simulink model "sm_car"  (R2025a)
settings: Solver=ode23t  StartTime=0.0  StopTime=400  MaxStep=0.4  RelTol=1e-3  AbsTol=1e-3  EnableMultiTasking=on
PreLoadFcn:
  | % Due to usability issue in Repeating Sequence block
  | warning('off','Simulink:Masking:Invalid');
  | 
  | % Eliminate unnecessary warnings in inactive variants
  | % Warnings generated only if you click through inactive variant
  | warning('off','MATLAB:nonExistentField');
  | warning('off','Simulink:Parameters:BlkParamUndefined');
PostLoadFcn:
  | set_param([bdroot '/Vehicle'],'popup_trailer','Off')
  | warning('off','sm:sli:setup:compile:LocalSolverNotSupported')
  | %sm_car_config_maneuver(bdroot,'WOT Braking');
  | sm_car_config_vehicle(bdroot,'false');
  | sm_car_config_logging(bdroot);
InitFcn:
  | sm_car_config_camera;
  | Vehicle = sm_car_vehcfg_checkConfig(Vehicle);
  | sm_car_check_tire_model(bdroot);
StartFcn:
  | tic;
StopFcn:
  | Elapsed_Sim_Time = toc;
  | % disp(['Elapsed Sim Time = ' num2str(Elapsed_Sim_Time)]);
undefined symbols (not defined in the file): Axle1D, AxleIn, Camera, Control, Driver, Free, Init, Maneuver, Pedal, RaceFix, RaceSpin, Scene, ShaftL1, ShaftL2, ShaftR1, ShaftR2, Soft, Stiff, Visual, X, xy_data_car_side, Y, Z
libraries: sm_lib x1546, nesl_utility x528, fl_lib x480, SimscapeFluids_lib x61, sdl_lib x49, simulink x29, ee_lib x7, simulink_extras x6, Linkage_Systems x4, Tire_1x2x x4, AntiRollBar_Systems x2, Linkage_Decoupled x2
(part 11 of 79)

== system sm_car/Vehicle/Vehicle/Chassis/SuspA1/Linkage Decoupled ==
  In Bus Element : Inport  PortName=CtrlBus  Element=Steer
  DrvBus : Inport  Port=2
  Linkage L : Linkage_Decoupled/Linkage  VariantControl=Variant1  LabelModeActiveChoice=DWDecoupled  popup_leftRight=Left  Linkage=Susp.Linkage  InitLinkage=Init  VariantLabel=Susp.Linkage.class.Value
      settings: AttributesFormatString=%<ActiveVariant>
  Linkage R : Linkage_Decoupled/Linkage  VariantControl=Variant1  LabelModeActiveChoice=DWDecoupled  popup_leftRight=Right  Linkage=Susp.Linkage  InitLinkage=Init  VariantLabel=Susp.Linkage.class.Value
      settings: AttributesFormatString=%<ActiveVariant>
  RollHeave Decouple : Subsystem  VariantControl=Variant1  mask(Roll and Heave Spring Dampers){hp_pushrod=Susp.Linkage.Pushrod.sBellcrank.Value, hp_bcr_pivot=Susp.Linkage.Bellcrank.sPivot.Value, hp_bcr_shock_heaveL=Susp.Linkage.Shock.Heave.sLeft.Value, hp_bcr_shock_heaveR=Susp.Linkage.Shock.Heave.sRight.Value, hp_bcr_shock_rollL=Susp.Linkage.Shock.Roll.sLeft.Value, hp_bcr_shock_rollR=Susp.Linkage.Shock.Roll.sRight.Value, shock_pist_mass_heave=Susp.Linkage.Shock.Heave.mPiston.Value, shock_pist_mass_roll=Susp.Linkage.Shock.Roll.mPiston.Value, shock_cyl_mass_heave=Susp.Linkage.Shock.Heave.mCylinder.Value, shock_cyl_mass_roll=Susp.Linkage.Shock.Roll.mCylinder.Value, up_lim_bumpstop_heave=Susp.Linkage.Endstop.Heave.xMax.Value, up_lim_bumpstop_roll=Susp.Linkage.Endstop.Roll.xMax.Value, low_lim_bumpstop_heave=Susp.Linkage.Endstop.Heave.xMin.Value, low_lim_bumpstop_roll=Susp.Linkage.Endstop.Roll.xMin.Value, clr_conn_shock=Visual.hp.clr, opc_conn_shock=Visual.hp.opc, size_conn_shock=Visual.hp.rad, clr_shock_cyl=Visual.Shock.cyl.clr, opc_shock_cyl=Visual.part.opc, radius_shock_cyl=Visual.Shock.cyl.rad, clr_shock_piston=Visual.Shock.piston.clr, opc_shock_piston=Visual.part.opc, clr_shock_bumpstop=Visual.Shock.bumpstop.clr, opc_shock_bumpstop=Visual.part.opc, deadvol_len_shock_cyl=Visual.Shock.dead_length, piston_len_shock=Visual.Shock.piston.len, cyl_cap_len_shock=Visual.Shock.cap.len, bumpstop_len_shock=Visual.Shock.bumpstop.len}
      mask prompts: hp_pushrod "HP Pushrod Inner  [xyz] (m)"; hp_bcr_pivot "HP Bellcrank Pivot [xyz] (m)"; deadvol_len_shock_cyl "Dead Volume Height (m)"; piston_len_shock "Piston Length (m)"; cyl_cap_len_shock "Cylinder Cap Length (m)"; bumpstop_len_shock "Bumpstop Length (m)"
      mask help: Models springs and dampers in a suspension design that decouples stiffness and damping for body roll and heave.
      mask init:
      | % Code to mirror hardpoint about vehicle xz plane
      | % and the plane defined by the bellcrank pivot axis
      | % and the y axis of the vehicle
      | % Code not used so that points can be specified independently
      | % Left here as a reference.
      | %{
      |  
      | a1 = atan2(hp_pushrod(1)-hp_bcr_pivot(1)   ,hp_pushrod(3)-hp_bcr_pivot(3));
      | a2 = atan2(hp_bcr_shock_roll(1)-hp_bcr_pivot(1),hp_bcr_shock_roll(3)-hp_bcr_pivot(3));
      | d_roll2piv = norm(hp_bcr_shock_roll([1 3])-hp_bcr_pivot([1 3]));
      | d_roll_mirror_axis = d_roll2piv*cos(a2-a1);
      | mirr_dx = d_roll_mirror_axis*sin(a1);
      | mirr_dz = d_roll_mirror_axis*cos(a1);
      | hp_bcr_shock_roll_r = ...
      |     [hp_bcr_shock_roll(1)-2*mirr_dx -hp_bcr_shock_roll(2) hp_bcr_shock_roll(3)-2*mirr_dz]
      | %}
      mask TypeOptions shock_pist_mass_heave: Shock Heave/shock_pist_mass
      mask TypeOptions shock_pist_mass_roll: Shock Roll/shock_pist_mass
      mask TypeOptions shock_cyl_mass_heave: Shock Heave/shock_cyl_mass
      mask TypeOptions shock_cyl_mass_roll: Shock Roll/shock_cyl_mass
      mask TypeOptions up_lim_bumpstop_heave: Shock Heave/up_lim_bumpstop
      mask TypeOptions up_lim_bumpstop_roll: Shock Roll/up_lim_bumpstop
      mask TypeOptions low_lim_bumpstop_heave: Shock Heave/low_lim_bumpstop
      mask TypeOptions low_lim_bumpstop_roll: Shock Roll/low_lim_bumpstop
      mask TypeOptions clr_conn_shock: Shock Heave/clr_conn_shock | Shock Roll/clr_conn_shock
      mask TypeOptions opc_conn_shock: Shock Heave/opc_conn_shock | Shock Roll/opc_conn_shock
      mask TypeOptions size_conn_shock: Shock Heave/size_conn_shock | Shock Roll/size_conn_shock
      mask TypeOptions clr_shock_cyl: Shock Heave/clr_shock_cyl | Shock Roll/clr_shock_cyl
      mask TypeOptions opc_shock_cyl: Shock Heave/opc_shock_cyl | Shock Roll/opc_shock_cyl
      mask TypeOptions radius_shock_cyl: Shock Heave/radius_shock_cyl | Shock Roll/radius_shock_cyl
      mask TypeOptions clr_shock_piston: Shock Heave/clr_shock_piston | Shock Roll/clr_shock_piston
      mask TypeOptions opc_shock_piston: Shock Heave/opc_shock_piston | Shock Roll/opc_shock_piston
      mask TypeOptions clr_shock_bumpstop: Shock Heave/clr_shock_bumpstop | Shock Roll/clr_shock_bumpstop
      mask TypeOptions opc_shock_bumpstop: Shock Heave/opc_shock_bumpstop | Shock Roll/opc_shock_bumpstop
      mask TypeOptions deadvol_len_shock_cyl: Shock Heave/deadvol_len_shock_cyl | Shock Roll/deadvol_len_shock_cyl
      mask TypeOptions piston_len_shock: Shock Heave/piston_len_shock | Shock Roll/piston_len_shock
      mask TypeOptions cyl_cap_len_shock: Shock Heave/cyl_cap_len_shock | Shock Roll/cyl_cap_len_shock
      mask TypeOptions bumpstop_len_shock: Shock Heave/bumpstop_len_shock | Shock Roll/bumpstop_len_shock
      mask DialogControl cont_hp Prompt: Hardpoints
      mask DialogControl text_hp_left Prompt: Left
      mask DialogControl text_hp_right Prompt: Right
      mask DialogControl text_hp_heave Prompt: Heave [xyz] (m)
      mask DialogControl text_hp_roll Prompt: Roll [xyz] (m)
      mask DialogControl cont_shock Prompt: Shock
      mask DialogControl text_shock_parts_blank Prompt: Parts
      mask DialogControl text_shock_heave Prompt: Heave
      mask DialogControl text_shock_roll Prompt: Roll
      mask DialogControl text_shock_pistm Prompt: Piston Mass (kg)
      mask DialogControl text_shock_cylm Prompt: Cylinder Mass (kg)
      mask DialogControl text_shock_bumpstop_par Prompt: Bumpstop
      mask DialogControl text_bump_ul Prompt: Upper Limit (m)
      mask DialogControl text_bump_low Prompt: Lower Limit (m)
      mask DialogControl cont_vis_shock Prompt: Visualization
      mask DialogControl text_clr_shock Prompt: Color  [RGB]
      mask DialogControl text_opc_shock Prompt: Opac. (0-1)
      mask DialogControl text_size_shock Prompt: Size (m)
      mask DialogControl text_conn_shock Prompt: Connections
      mask DialogControl text_shock_shock Prompt: Cylinder
      mask DialogControl text_shock_piston Prompt: Piston
      mask DialogControl text_piston_radius Prompt: <cylinder radius>
      mask DialogControl text_shock_bumpstop Prompt: Bumpstop
      mask DialogControl text_bumpstop_radius Prompt: <cylinder radius>
      mask Display: image('sm_car_vehicle_linkage_rollHeaveDecouple_IMAGE.png');
  Simscape Bus L : SimscapeBus  HierarchyStrings=RaceSpin;RaceFix;Axle1D;AxleIn
  Simscape Bus L1 : SimscapeBus  HierarchyStrings=RaceSpin;RaceFix;Axle1D;AxleIn
  Steer : Subsystem  Variant=on  VariantControlMode=label  VariantControl=Steer  LabelModeActiveChoice=WheelDrivenRack1UJoint  mask(Steering System with Rack){Steer=Susp.Steer, VariantLabel=Susp.Steer.class.Value}
      mask prompts: Steer "Steer Parameters"; VariantLabel "Variant Label"
      mask help: Models steering system that involves a rack. Optionally include steering wheel. Connection between steering wheel and rack can be mechanical, specified by a lookup table, or a control system as in steer-by-wire. Option is chosen by string provided in Variant Label. The parameters for the selected option are contained in Steer data structure.
      mask init:
      | curblk = gcb;
      | 
      | % Set variant for this block 
      | set_param(curblk,'LabelModeActiveChoice',VariantLabel);
      settings: AttributesFormatString=%<ActiveVariant>
      mask Display: disp(' ');
  Wheel Meas Left : Subsystem  mask(Wheel Measurements){popup_leftRight=Left}
      mask prompts: popup_leftRight "Left/Right"
      mask help: Calculates toe and camber angles based on orientation of wheel spin axis. To estimate steering axis inclination, the same measurements are done along the longitudinal axis (X) of the tire. Set Left/Right so that the sign of the logged toe and camber angles is associated with towards/away from vehicle center.
      mask init:
      | if(popup_leftRight == 1)
      |     rhs_tc = 1;
      | elseif(popup_leftRight == 2)
      |     rhs_tc = -1;
      | end
      mask TypeOptions popup_leftRight: Left | Right
  Wheel Meas Right : Subsystem  mask(Wheel Measurements){popup_leftRight=Right}
      mask prompts: popup_leftRight "Left/Right"
      mask help: Calculates toe and camber angles based on orientation of wheel spin axis. To estimate steering axis inclination, the same measurements are done along the longitudinal axis (X) of the tire. Set Left/Right so that the sign of the logged toe and camber angles is associated with towards/away from vehicle center.
      mask init:
      | if(popup_leftRight == 1)
      |     rhs_tc = 1;
      | elseif(popup_leftRight == 2)
      |     rhs_tc = -1;
      | end
      mask TypeOptions popup_leftRight: Left | Right
  WCL : PMIOPort  Side=Left
  Ref : PMIOPort  Port=2  Side=Right
  WCR : PMIOPort  Port=3  Side=Right
  AxleL : PMIOPort  Port=4  Side=Left
  AxleR : PMIOPort  Port=5  Side=Right
  SprL : PMIOPort  Port=6  Side=Left
  SprR : PMIOPort  Port=7  Side=Right
  DmpL : PMIOPort  Port=8  Side=Left
  DmpR : PMIOPort  Port=9  Side=Right
  Out Bus Element : Outport  VectorParamsAs1DForOutWhenUnconnected=off  PortName=OutBus  Element=Steer
  Out Bus Element1 : Outport  VectorParamsAs1DForOutWhenUnconnected=off  PortName=OutBus  Element=RollHeave
  Out Bus Element2 : Outport  VectorParamsAs1DForOutWhenUnconnected=off  PortName=OutBus  Element=WhlL
  Out Bus Element3 : Outport  VectorParamsAs1DForOutWhenUnconnected=off  PortName=OutBus  Element=WhlR
  Out Bus Element4 : Outport  VectorParamsAs1DForOutWhenUnconnected=off  PortName=OutBus  Element=LinkageR
  Out Bus Element5 : Outport  VectorParamsAs1DForOutWhenUnconnected=off  PortName=OutBus  Element=LinkageL
  wires:
  Linkage L/1 -> Out Bus Element5/1
  Linkage R/1 -> Out Bus Element4/1
  RollHeave Decouple/1(meas) -> Out Bus Element1/1
  DrvBus/1 -> Steer/1(DrvBus)
  Steer/1(" meas") -> Out Bus Element/1
  In Bus Element/1 -> Steer/2(CtrlBus)
  Wheel Meas Left/1(meas) -> Out Bus Element2/1
  Wheel Meas Right/1(meas) -> Out Bus Element3/1
  connections:
  SprR/RConn1 -- RollHeave Decouple/LConn5
  DmpR/RConn1 -- RollHeave Decouple/LConn6
  SprL/RConn1 -- RollHeave Decouple/LConn3
  DmpL/RConn1 -- RollHeave Decouple/LConn4
  RollHeave Decouple/LConn8 -- Linkage R/LConn6
  RollHeave Decouple/LConn7 -- Linkage R/LConn7
  RollHeave Decouple/LConn2 -- Linkage L/LConn7
  Steer/RConn3 -- Linkage R/RConn1
  Linkage L/RConn2 -- Ref/RConn1 -- Linkage R/RConn2 -- Wheel Meas Left/LConn1 -- Wheel Meas Right/LConn1 -- Steer/RConn2
  WCL/RConn1 -- Linkage L/LConn1 -- Wheel Meas Left/LConn2
  WCR/RConn1 -- Linkage R/LConn1 -- Wheel Meas Right/LConn2
  Steer/RConn1 -- Linkage L/RConn1
  Linkage L/LConn5 -- Simscape Bus L/LConn4
  Linkage L/LConn2 -- Simscape Bus L/LConn1
  Linkage L/LConn3 -- Simscape Bus L/LConn2
  Linkage L/LConn4 -- Simscape Bus L/LConn3
  AxleL/RConn1 -- Simscape Bus L/RConn1
  Linkage R/LConn2 -- Simscape Bus L1/LConn1
  Linkage R/LConn3 -- Simscape Bus L1/LConn2
  Linkage R/LConn4 -- Simscape Bus L1/LConn3
  Simscape Bus L1/RConn1 -- AxleR/RConn1
  Linkage R/LConn5 -- Simscape Bus L1/LConn4
  RollHeave Decouple/LConn1 -- Linkage L/LConn6

== system sm_car/Vehicle/Vehicle/Chassis/SuspA2/Linkage ==
  In Bus Element : Inport  PortName=CtrlBus  Element=Steer
  DrvBus : Inport  Port=2
  Anti Roll Bar : AntiRollBar_Systems/Anti Roll Bar  LabelModeActiveChoice=DroplinkRod  AntiRollBar=Susp.AntiRollBar  VariantLabel=Susp.AntiRollBar.class.Value
      settings: AttributesFormatString=%<LabelModeActiveChoice>
  Linkage L : Linkage_Systems/Linkage  VariantControl=Variant1  LabelModeActiveChoice=DoubleWishboneA  popup_leftRight=Left  Linkage=Susp.Linkage  InitLinkage=Init  VariantLabel=Susp.Linkage.class.Value
      settings: AttributesFormatString=%<ActiveVariant>
  Linkage R : Linkage_Systems/Linkage  Tag=PublishSubsystem  VariantControl=Variant1  LabelModeActiveChoice=DoubleWishboneA  popup_leftRight=Right  Linkage=Susp.Linkage  InitLinkage=Init  VariantLabel=Susp.Linkage.class.Value
      settings: AttributesFormatString=%<ActiveVariant>
  Simscape Bus L : SimscapeBus  HierarchyStrings=RaceSpin;RaceFix;Axle1D;AxleIn
  Simscape Bus L1 : SimscapeBus  HierarchyStrings=RaceSpin;RaceFix;Axle1D;AxleIn
  Steer : Subsystem  Variant=on  VariantControlMode=label  VariantControl=Steer  LabelModeActiveChoice=None  mask(Steering System with Rack){Steer=Susp.Steer, VariantLabel=Susp.Steer.class.Value}
      mask prompts: Steer "Steer Parameters"; VariantLabel "Variant Label"
      mask help: Models steering system that involves a rack. Optionally include steering wheel. Connection between steering wheel and rack can be mechanical, specified by a lookup table, or a control system as in steer-by-wire. Option is chosen by string provided in Variant Label. The parameters for the selected option are contained in Steer data structure.
      mask init:
      | curblk = gcb;
      | 
      | % Set variant for this block 
      | set_param(curblk,'LabelModeActiveChoice',VariantLabel);
      settings: AttributesFormatString=%<ActiveVariant>
      mask Display: disp(' ');
  Wheel Meas Left : Subsystem  mask(Wheel Measurements){popup_leftRight=Left}
      mask prompts: popup_leftRight "Left/Right"
      mask help: Calculates toe and camber angles based on orientation of wheel spin axis. To estimate steering axis inclination, the same measurements are done along the longitudinal axis (X) of the tire. Set Left/Right so that the sign of the logged toe and camber angles is associated with towards/away from vehicle center.
      mask init:
      | if(popup_leftRight == 1)
      |     rhs_tc = 1;
      | elseif(popup_leftRight == 2)
      |     rhs_tc = -1;
      | end
      mask TypeOptions popup_leftRight: Left | Right
  Wheel Meas Right : Subsystem  mask(Wheel Measurements){popup_leftRight=Right}
      mask prompts: popup_leftRight "Left/Right"
      mask help: Calculates toe and camber angles based on orientation of wheel spin axis. To estimate steering axis inclination, the same measurements are done along the longitudinal axis (X) of the tire. Set Left/Right so that the sign of the logged toe and camber angles is associated with towards/away from vehicle center.
      mask init:
      | if(popup_leftRight == 1)
      |     rhs_tc = 1;
      | elseif(popup_leftRight == 2)
      |     rhs_tc = -1;
      | end
      mask TypeOptions popup_leftRight: Left | Right
  WCL : PMIOPort  Side=Left
  Ref : PMIOPort  Port=2  Side=Right
  WCR : PMIOPort  Port=3  Side=Right
  AxleL : PMIOPort  Port=4  Side=Left
  AxleR : PMIOPort  Port=5  Side=Right
  SprL : PMIOPort  Port=6  Side=Left
  SprR : PMIOPort  Port=7  Side=Right
  DmpL : PMIOPort  Port=8  Side=Left
  DmpR : PMIOPort  Port=9  Side=Right
  Out Bus Element : Outport  VectorParamsAs1DForOutWhenUnconnected=off  PortName=OutBus  Element=Steer
  Out Bus Element1 : Outport  VectorParamsAs1DForOutWhenUnconnected=off  PortName=OutBus  Element=AntiRollBar
  Out Bus Element2 : Outport  VectorParamsAs1DForOutWhenUnconnected=off  PortName=OutBus  Element=WhlL
  Out Bus Element3 : Outport  VectorParamsAs1DForOutWhenUnconnected=off  PortName=OutBus  Element=WhlR
  Out Bus Element4 : Outport  VectorParamsAs1DForOutWhenUnconnected=off  PortName=OutBus  Element=LinkageR
  Out Bus Element5 : Outport  VectorParamsAs1DForOutWhenUnconnected=off  PortName=OutBus  Element=LinkageL
  wires:
  Linkage L/1 -> Out Bus Element5/1
  Linkage R/1 -> Out Bus Element4/1
  DrvBus/1 -> Steer/1(DrvBus)
  Steer/1(" meas") -> Out Bus Element/1
  In Bus Element/1 -> Steer/2(CtrlBus)
  Anti Roll Bar/1 -> Out Bus Element1/1
  Wheel Meas Left/1(meas) -> Out Bus Element2/1
  Wheel Meas Right/1(meas) -> Out Bus Element3/1
  connections:
  Steer/RConn3 -- Linkage R/RConn1
  Ref/RConn1 -- Anti Roll Bar/LConn2 -- Linkage R/RConn2 -- Wheel Meas Right/LConn1 -- Wheel Meas Left/LConn1 -- Steer/RConn2 -- Linkage L/RConn2
  Linkage L/LConn1 -- WCL/RConn1 -- Wheel Meas Left/LConn2
  Linkage R/LConn1 -- WCR/RConn1 -- Wheel Meas Right/LConn2
  Steer/RConn1 -- Linkage L/RConn1
  DmpL/RConn1 -- Linkage L/LConn7
  Simscape Bus L/LConn4 -- Linkage L/LConn5
  Simscape Bus L/LConn1 -- Linkage L/LConn2
  Linkage L/LConn3 -- Simscape Bus L/LConn2
  Linkage L/LConn4 -- Simscape Bus L/LConn3
  AxleL/RConn1 -- Simscape Bus L/RConn1
  DmpR/RConn1 -- Linkage R/LConn7
  SprR/RConn1 -- Linkage R/LConn6
  Simscape Bus L1/LConn1 -- Linkage R/LConn2
  Simscape Bus L1/LConn2 -- Linkage R/LConn3
  Simscape Bus L1/LConn3 -- Linkage R/LConn4
  Simscape Bus L1/RConn1 -- AxleR/RConn1
  SprL/RConn1 -- Linkage L/LConn6
  Simscape Bus L1/LConn4 -- Linkage R/LConn5
  Anti Roll Bar/LConn3 -- Linkage R/LConn8
  Anti Roll Bar/LConn1 -- Linkage L/LConn8

== system sm_car/Vehicle/Vehicle/Powertrain/Driveline/L1 R1 L2 R2 ==
  note: Port
      | placement
  In Bus Element1 : Inport  PortName=CtrlBus
  Gearbox L1 : sdl_lib/Gears/Simple Gear  ratio=Driveline.GearboxL1.ratio.Value  rotation_direction=3-2*(1)  friction_model=1  T_noload=0.1 N*m  T_nom=5 N*m  efficiency_nom=0.8  efficiency=0.8  temperature_TLU=[280, 300, 320] K  load_TLU=[1, 5, 10] N*m  efficiency_TLU=[.95, .9, .85]  efficiency_TLU2=[.85, .8, .75; .95, .9, .85; .85, .8, .7]  w_thr=0.01 rad/s  pwr_thr=0.001 W  enable_backlash=false  hardstop_model=simscape.enum.hardstop.smooth  backlash_distance=1e-3 mm  r_base=0.1 m  transition=1e-4 mm  backlash_stiffness=1e7 N/m  backlash_damping=1e6 N*s/m  coeff_rest=0  v_tol=0.001 m/s  f_tol=0 N  mu_visc=[0, 0] N*m/(rad/s)  thermal_mass=50 J/K  temperature_specify=off  temperature_priority=High  temperature=300 K  temperature_nominal_specify=off  temperature_nominal_value=1  temperature_nominal_unit=K  x_backlash_specify=off  x_backlash_priority=None  x_backlash=0 mm  x_backlash_nominal_specify=off  x_backlash_nominal_value=1  x_backlash_nominal_unit=mm  f_hardstop_specify=off  f_hardstop_priority=None  f_hardstop=0 N  f_hardstop_nominal_specify=off  f_hardstop_nominal_value=1  f_hardstop_nominal_unit=N  v_backlash_specify=off  v_backlash_priority=None  v_backlash=0 m/s  v_backlash_nominal_specify=off  v_backlash_nominal_value=1  v_backlash_nominal_unit=m/s
  Gearbox L2 : sdl_lib/Gears/Simple Gear  ratio=Driveline.GearboxL2.ratio.Value  rotation_direction=3-2*(1)  friction_model=1  T_noload=0.1 N*m  T_nom=5 N*m  efficiency_nom=0.8  efficiency=0.8  temperature_TLU=[280, 300, 320] K  load_TLU=[1, 5, 10] N*m  efficiency_TLU=[.95, .9, .85]  efficiency_TLU2=[.85, .8, .75; .95, .9, .85; .85, .8, .7]  w_thr=0.01 rad/s  pwr_thr=0.001 W  enable_backlash=false  hardstop_model=simscape.enum.hardstop.smooth  backlash_distance=1e-3 mm  r_base=0.1 m  transition=1e-4 mm  backlash_stiffness=1e7 N/m  backlash_damping=1e6 N*s/m  coeff_rest=0  v_tol=0.001 m/s  f_tol=0 N  mu_visc=[0, 0] N*m/(rad/s)  thermal_mass=50 J/K  temperature_specify=off  temperature_priority=High  temperature=300 K  temperature_nominal_specify=off  temperature_nominal_value=1  temperature_nominal_unit=K  x_backlash_specify=off  x_backlash_priority=None  x_backlash=0 mm  x_backlash_nominal_specify=off  x_backlash_nominal_value=1  x_backlash_nominal_unit=mm  f_hardstop_specify=off  f_hardstop_priority=None  f_hardstop=0 N  f_hardstop_nominal_specify=off  f_hardstop_nominal_value=1  f_hardstop_nominal_unit=N  v_backlash_specify=off  v_backlash_priority=None  v_backlash=0 m/s  v_backlash_nominal_specify=off  v_backlash_nominal_value=1  v_backlash_nominal_unit=m/s
  Gearbox R1 : sdl_lib/Gears/Simple Gear  ratio=Driveline.GearboxL1.ratio.Value  rotation_direction=3-2*(1)  friction_model=1  T_noload=0.1 N*m  T_nom=5 N*m  efficiency_nom=0.8  efficiency=0.8  temperature_TLU=[280, 300, 320] K  load_TLU=[1, 5, 10] N*m  efficiency_TLU=[.95, .9, .85]  efficiency_TLU2=[.85, .8, .75; .95, .9, .85; .85, .8, .7]  w_thr=0.01 rad/s  pwr_thr=0.001 W  enable_backlash=false  hardstop_model=simscape.enum.hardstop.smooth  backlash_distance=1e-3 mm  r_base=0.1 m  transition=1e-4 mm  backlash_stiffness=1e7 N/m  backlash_damping=1e6 N*s/m  coeff_rest=0  v_tol=0.001 m/s  f_tol=0 N  mu_visc=[0, 0] N*m/(rad/s)  thermal_mass=50 J/K  temperature_specify=off  temperature_priority=High  temperature=300 K  temperature_nominal_specify=off  temperature_nominal_value=1  temperature_nominal_unit=K  x_backlash_specify=off  x_backlash_priority=None  x_backlash=0 mm  x_backlash_nominal_specify=off  x_backlash_nominal_value=1  x_backlash_nominal_unit=mm  f_hardstop_specify=off  f_hardstop_priority=None  f_hardstop=0 N  f_hardstop_nominal_specify=off  f_hardstop_nominal_value=1  f_hardstop_nominal_unit=N  v_backlash_specify=off  v_backlash_priority=None  v_backlash=0 m/s  v_backlash_nominal_specify=off  v_backlash_nominal_value=1  v_backlash_nominal_unit=m/s
  Gearbox R2 : sdl_lib/Gears/Simple Gear  ratio=Driveline.GearboxR2.ratio.Value  rotation_direction=3-2*(1)  friction_model=1  T_noload=0.1 N*m  T_nom=5 N*m  efficiency_nom=0.8  efficiency=0.8  temperature_TLU=[280, 300, 320] K  load_TLU=[1, 5, 10] N*m  efficiency_TLU=[.95, .9, .85]  efficiency_TLU2=[.85, .8, .75; .95, .9, .85; .85, .8, .7]  w_thr=0.01 rad/s  pwr_thr=0.001 W  enable_backlash=false  hardstop_model=simscape.enum.hardstop.smooth  backlash_distance=1e-3 mm  r_base=0.1 m  transition=1e-4 mm  backlash_stiffness=1e7 N/m  backlash_damping=1e6 N*s/m  coeff_rest=0  v_tol=0.001 m/s  f_tol=0 N  mu_visc=[0, 0] N*m/(rad/s)  thermal_mass=50 J/K  temperature_specify=off  temperature_priority=High  temperature=300 K  temperature_nominal_specify=off  temperature_nominal_value=1  temperature_nominal_unit=K  x_backlash_specify=off  x_backlash_priority=None  x_backlash=0 mm  x_backlash_nominal_specify=off  x_backlash_nominal_value=1  x_backlash_nominal_unit=mm  f_hardstop_specify=off  f_hardstop_priority=None  f_hardstop=0 N  f_hardstop_nominal_specify=off  f_hardstop_nominal_value=1  f_hardstop_nominal_unit=N  v_backlash_specify=off  v_backlash_priority=None  v_backlash=0 m/s  v_backlash_nominal_specify=off  v_backlash_nominal_value=1  v_backlash_nominal_unit=m/s
  Reference Frame : sm_lib/Frames and Transforms/Reference Frame
  Reference Frame1 : sm_lib/Frames and Transforms/Reference Frame
  Sensing Torque L1 : Subsystem
  Sensing Torque L2 : Subsystem
  Sensing Torque R1 : Subsystem
  Sensing Torque R2 : Subsystem
  ShaftL1 : Subsystem  VariantControl=Shaft1D  mask(Driveshaft Assembly (1D)){}
      mask help: Models a shaft as a 1D mechanical connection.
  ShaftL2 : Subsystem  VariantControl=Shaft1D  mask(Driveshaft Assembly (1D)){}
      mask help: Models a shaft as a 1D mechanical connection.
  ShaftR1 : Subsystem  VariantControl=Shaft1D  mask(Driveshaft Assembly (1D)){}
      mask help: Models a shaft as a 1D mechanical connection.
  ShaftR2 : Subsystem  VariantControl=Shaft1D  mask(Driveshaft Assembly (1D)){}
      mask help: Models a shaft as a 1D mechanical connection.
  Simscape Bus : SimscapeBus  HierarchyStrings=ShaftL1;ShaftR1;ShaftR2;ShaftL2
  Simscape L1 : SimscapeBus  HierarchyStrings=Shaft1D
  Simscape L2 : SimscapeBus  HierarchyStrings=Shaft1D
  Simscape R1 : SimscapeBus  HierarchyStrings=Shaft1D
  Simscape R2 : SimscapeBus  HierarchyStrings=Shaft1D
  Terminator : Terminator
  A1 : PMIOPort  Side=Left
  A2 : PMIOPort  Port=2  Side=Right
  L1 : PMIOPort  Port=3  Side=Left
  R1 : PMIOPort  Port=4  Side=Right
  L2 : PMIOPort  Port=5  Side=Left
  R2 : PMIOPort  Port=6  Side=Right
  Shafts : PMIOPort  Port=7  Side=Left
  o : PMIOPort  Port=8  Side=Right
  Out Bus Element6 : Outport  VectorParamsAs1DForOutWhenUnconnected=off  PortName=OutD  Element=MDriveshaftL2
  Out Bus Element7 : Outport  VectorParamsAs1DForOutWhenUnconnected=off  PortName=OutD  Element=MDriveshaftR2
  Out Bus Element4 : Outport  VectorParamsAs1DForOutWhenUnconnected=off  PortName=OutD  Element=MDriveshaftR1
  Out Bus Element5 : Outport  VectorParamsAs1DForOutWhenUnconnected=off  PortName=OutD  Element=MDriveshaftL1
  Out Bus Element : Outport  VectorParamsAs1DForOutWhenUnconnected=off  PortName=OutD  Element=anDriveshaftL1
  Out Bus Element1 : Outport  VectorParamsAs1DForOutWhenUnconnected=off  PortName=OutD  Element=anDriveshaftR1
  Out Bus Element2 : Outport  VectorParamsAs1DForOutWhenUnconnected=off  PortName=OutD  Element=anDriveshaftL2
  Out Bus Element3 : Outport  VectorParamsAs1DForOutWhenUnconnected=off  PortName=OutD  Element=anDriveshaftR2
  wires:
  ShaftR1/1(meas) -> Out Bus Element1/1
  ShaftL1/1(meas) -> Out Bus Element/1
  ShaftL2/1(meas) -> Out Bus Element2/1
  ShaftR2/1(meas) -> Out Bus Element3/1
  Sensing Torque R2/1(M) -> Out Bus Element7/1
  Sensing Torque L2/1(M) -> Out Bus Element6/1
  Sensing Torque R1/1(M) -> Out Bus Element4/1
  Sensing Torque L1/1(M) -> Out Bus Element5/1
  In Bus Element1/1 -> Terminator/1
  connections:
  Gearbox L2/RConn1 -- Sensing Torque L2/LConn1
  Sensing Torque R2/LConn1 -- Gearbox R2/RConn1
  Simscape L1/LConn1 -- Sensing Torque L1/RConn1
  Sensing Torque R1/RConn1 -- Simscape R1/LConn1
  Sensing Torque R1/LConn1 -- Gearbox R1/RConn1
  Gearbox R1/LConn1 -- Simscape Bus/LConn2 -- o/RConn1
  A1/RConn1 -- Reference Frame1/RConn1
  ShaftL1/RConn1 -- Simscape L1/RConn1
  Gearbox L1/RConn1 -- Sensing Torque L1/LConn1
  Simscape Bus/LConn3 -- Gearbox R2/LConn1
  Gearbox L2/LConn1 -- Simscape Bus/LConn4
  Simscape L2/LConn1 -- Sensing Torque L2/RConn1
  Simscape L2/RConn1 -- ShaftL2/RConn1
  Gearbox L1/LConn1 -- Simscape Bus/LConn1
  ShaftR1/RConn1 -- Simscape R1/RConn1
  ShaftR1/LConn1 -- R1/RConn1
  ShaftL1/LConn1 -- L1/RConn1
  Reference Frame/RConn1 -- A2/RConn1
  ShaftR2/LConn1 -- R2/RConn1
  ShaftL2/LConn1 -- L2/RConn1
  Simscape R2/RConn1 -- ShaftR2/RConn1
  Sensing Torque R2/RConn1 -- Simscape R2/LConn1
  Simscape Bus/RConn1 -- Shafts/RConn1

== system sm_car/Vehicle/Vehicle/Powertrain/Power/Electric L1 R1 L2 R2 ==
  note: Future:
      | react torque
      | from drive
      | on chassis
  In Bus Element1 : Inport  PortName=CtrlBus  Element=MMotorL1Demand
  In Bus Element2 : Inport  PortName=CtrlBus  Element=MMotorL2Demand
  In Bus Element3 : Inport  PortName=CtrlBus  Element=MMotorR2Demand
  In Bus Element4 : Inport  PortName=CtrlBus  Element=MMotorR1Demand
  VehBus : Inport  Port=2
  Ambient Temperature : fl_lib/Thermal/Thermal Sources/Temperature Source  temperature=Power.TAmbient.Value K
  Battery : Subsystem
      mask Display: image('sm_car_vehicle_power_battery_system_IMAGE.png');
  ERef DC Bus : fl_lib/Electrical/Electrical Elements/Electrical Reference
  Motor L1 : Subsystem  mask(Motor and Drive){Motor=Power.MotorL1}
      mask prompts: Motor "Motor (Structure)"
      mask help: Models generic motor and drive with closed-loop torque control. Specify torque-speed curve and other parameters in the Motor data structure.
      mask Display: image('sm_car_vehicle_power_emotor_simplified_IMAGE.png');
  Motor L2 : Subsystem  mask(Motor and Drive){Motor=Power.MotorL2}
      mask prompts: Motor "Motor (Structure)"
      mask help: Models generic motor and drive with closed-loop torque control. Specify torque-speed curve and other parameters in the Motor data structure.
      mask Display: image('sm_car_vehicle_power_emotor_simplified_IMAGE.png');
  Motor R1 : Subsystem  mask(Motor and Drive){Motor=Power.MotorL1}
      mask prompts: Motor "Motor (Structure)"
      mask help: Models generic motor and drive with closed-loop torque control. Specify torque-speed curve and other parameters in the Motor data structure.
      mask Display: image('sm_car_vehicle_power_emotor_simplified_IMAGE.png');
  Motor R2 : Subsystem  mask(Motor and Drive){Motor=Power.MotorL2}
      mask prompts: Motor "Motor (Structure)"
      mask help: Models generic motor and drive with closed-loop torque control. Specify torque-speed curve and other parameters in the Motor data structure.
      mask Display: image('sm_car_vehicle_power_emotor_simplified_IMAGE.png');
  Reference Frame : sm_lib/Frames and Transforms/Reference Frame
  Simscape Bus : SimscapeBus  HierarchyStrings=ShaftL1;ShaftR1;ShaftL2;ShaftR2
  Terminator : Terminator
  Thermal : Subsystem  Variant=on  VariantControlMode=label  VariantControl=Variant1  LabelModeActiveChoice=Liquid_Loop1  mask(Variants for Cooling System){VariantLabel=Power.Cooling.class.Value}
      mask prompts: VariantLabel "Variant Label"
      mask help: Select option and provide parameters for cooling system. Option is chosen by string provided in Variant Label.
      mask init:
      | curblk = gcb;
      | 
      | % Set variant for this block 
      | set_param(curblk,'LabelModeActiveChoice',VariantLabel);
      settings: AttributesFormatString=%<ActiveVariant>
  Shafts : PMIOPort  Side=Left
  Ref : PMIOPort  Port=2  Side=Right
  Out Bus Element : Outport  VectorParamsAs1DForOutWhenUnconnected=off  PortName=OutP  Element=MotorL2
  Out Bus Element1 : Outport  VectorParamsAs1DForOutWhenUnconnected=off  PortName=OutP  Element=MotorR2
  Out Bus Element2 : Outport  VectorParamsAs1DForOutWhenUnconnected=off  PortName=OutP  Element=MotorL1
  Out Bus Element3 : Outport  VectorParamsAs1DForOutWhenUnconnected=off  PortName=OutP  Element=Thermal
  Out Bus Element4 : Outport  VectorParamsAs1DForOutWhenUnconnected=off  PortName=OutP  Element=Battery
  Out Bus Element5 : Outport  VectorParamsAs1DForOutWhenUnconnected=off  PortName=OutP  Element=MotorR1
  wires:
  In Bus Element4/1 -> Motor R1/1(Tr)
  Motor R1/1(m) -> Out Bus Element5/1
  Battery/1(m) -> Out Bus Element4/1
  VehBus/1 -> Terminator/1
  Thermal/1(" m") -> Out Bus Element3/1
  In Bus Element3/1 -> Motor R2/1(Tr)
  Motor L1/1(m) -> Out Bus Element2/1
  Motor R2/1(m) -> Out Bus Element1/1
  Motor L2/1(m) -> Out Bus Element/1
  In Bus Element1/1 -> Motor L1/1(Tr)
  In Bus Element2/1 -> Motor L2/1(Tr)
  connections:
  Motor R1/LConn3 -- Thermal/LConn3
  Motor R1/RConn1 -- Simscape Bus/LConn2
  Thermal/RConn1 -- Battery/LConn1
  Battery/RConn3 -- Thermal/LConn1
  Thermal/RConn2 -- Ambient Temperature/LConn1
  Motor R2/LConn3 -- Thermal/LConn5
  Motor L2/LConn3 -- Thermal/LConn4
  Motor L1/LConn3 -- Thermal/LConn2
  Ref/RConn1 -- Reference Frame/RConn1
  Simscape Bus/RConn1 -- Shafts/RConn1
  Motor L2/RConn1 -- Simscape Bus/LConn3
  Motor L1/RConn1 -- Simscape Bus/LConn1
  Motor R2/LConn1 -- Motor L1/LConn1 -- Battery/RConn1 -- Motor R1/LConn1 -- Motor L2/LConn1
  Motor L1/LConn2 -- Battery/RConn2 -- Motor R1/LConn2 -- ERef DC Bus/LConn1 -- Motor R2/LConn2 -- Motor L2/LConn2
  Motor R2/RConn1 -- Simscape Bus/LConn4

== system sm_car/World/Scene/CRG Hockenheim/Finish Line/L1 ==
  Square LL : sm_lib/Body Elements/Brick Solid  BrickDimensions=square_lwh  BrickDimensionsUnits=m  ExportEntireGeometry=off  InertiaType=CalculateFromGeometry  BasedOnType=Density  Density=1000  DensityUnits=kg/m^3  Mass=1  MassUnits=kg  CenterOfMass=[0 0 0]  CenterOfMassUnits=m  MomentsOfInertia=[1 1 1]  MomentsOfInertiaUnits=kg*m^2  ProductsOfInertia=[0 0 0]  ProductsOfInertiaUnits=kg*m^2  GraphicType=FromGeometry  MarkerShape=Sphere  MarkerSize=10  GraphicVisPropType=SimpleVisualProperties  GraphicDiffuseColor=[0.0 0.0 0.0]  GraphicOpacity=1.0  GraphicSpecularColor=[0.5 0.5 0.5 1.0]  GraphicAmbientColor=[0.15 0.15 0.15 1.0]  GraphicEmissiveColor=[0.0 0.0 0.0 1.0]  GraphicShininess=75  DoExposeReferenceFrame=off  SerializedFrames=<Frames><Frame><Id>Frame1</Id><Value><Name>BL</Name><Origin><Source>GeometricFeature</Source><FeatureName>+y -z curve</FeatureName></Origin><PrimaryAxis><DefinedDirection>+Z</DefinedDirection><Source>ReferenceFrame</Source><SourceDirection>+Z</SourceDirection><FeatureName></FeatureName></PrimaryAxis><SecondaryAxis><DefinedDirection>+X</DefinedDirection><Source>ReferenceFrame</Source><SourceDirection>+X</SourceDirection><FeatureName></FeatureName></SecondaryAxis></Value></Frame><Frame><Id>Frame2</Id><Value><Name>TL</Name><Origin><Source>GeometricFeature</Source><FeatureName>+x +y +z point</FeatureName></Origin><PrimaryAxis><DefinedDirection>+Z</DefinedDirection><Source>ReferenceFrame</Source><SourceDirection>+Z</SourceDirection><FeatureName></FeatureName></PrimaryAxis><SecondaryAxis><DefinedDirection>+X</DefinedDirection><Source>ReferenceFrame</Source><SourceDirection>+X</SourceDirection><FeatureName></FeatureName></SecondaryAxis></Value></Frame><Frame><Id>Frame3</Id><Value><Name>BR</Name><Origin><Source>GeometricFeature</Source><FeatureName>-y -z curve</FeatureName></Origin><PrimaryAxis><DefinedDirection>+Z</DefinedDirection><Source>ReferenceFrame</Source><SourceDirection>+Z</SourceDirection><FeatureName></FeatureName></PrimaryAxis><SecondaryAxis><DefinedDirection>+X</DefinedDirection><Source>ReferenceFrame</Source><SourceDirection>+X</SourceDirection><FeatureName></FeatureName></SecondaryAxis></Value></Frame></Frames>
  Square LR : sm_lib/Body Elements/Brick Solid  BrickDimensions=square_lwh  BrickDimensionsUnits=m  ExportEntireGeometry=off  InertiaType=CalculateFromGeometry  BasedOnType=Density  Density=1000  DensityUnits=kg/m^3  Mass=1  MassUnits=kg  CenterOfMass=[0 0 0]  CenterOfMassUnits=m  MomentsOfInertia=[1 1 1]  MomentsOfInertiaUnits=kg*m^2  ProductsOfInertia=[0 0 0]  ProductsOfInertiaUnits=kg*m^2  GraphicType=FromGeometry  MarkerShape=Sphere  MarkerSize=10  GraphicVisPropType=SimpleVisualProperties  GraphicDiffuseColor=[1.0 1.0 1.0]  GraphicOpacity=1.0  GraphicSpecularColor=[0.5 0.5 0.5 1.0]  GraphicAmbientColor=[0.15 0.15 0.15 1.0]  GraphicEmissiveColor=[0.0 0.0 0.0 1.0]  GraphicShininess=75  DoExposeReferenceFrame=off  SerializedFrames=<Frames><Frame><Id>Frame1</Id><Value><Name>BL</Name><Origin><Source>GeometricFeature</Source><FeatureName>+y -z curve</FeatureName></Origin><PrimaryAxis><DefinedDirection>+Z</DefinedDirection><Source>ReferenceFrame</Source><SourceDirection>+Z</SourceDirection><FeatureName></FeatureName></PrimaryAxis><SecondaryAxis><DefinedDirection>+X</DefinedDirection><Source>ReferenceFrame</Source><SourceDirection>+X</SourceDirection><FeatureName></FeatureName></SecondaryAxis></Value></Frame><Frame><Id>Frame2</Id><Value><Name>TL</Name><Origin><Source>GeometricFeature</Source><FeatureName>+x +y +z point</FeatureName></Origin><PrimaryAxis><DefinedDirection>+Z</DefinedDirection><Source>ReferenceFrame</Source><SourceDirection>+Z</SourceDirection><FeatureName></FeatureName></PrimaryAxis><SecondaryAxis><DefinedDirection>+X</DefinedDirection><Source>ReferenceFrame</Source><SourceDirection>+X</SourceDirection><FeatureName></FeatureName></SecondaryAxis></Value></Frame><Frame><Id>Frame3</Id><Value><Name>BR</Name><Origin><Source>GeometricFeature</Source><FeatureName>-y -z curve</FeatureName></Origin><PrimaryAxis><DefinedDirection>+Z</DefinedDirection><Source>ReferenceFrame</Source><SourceDirection>+Z</SourceDirection><FeatureName></FeatureName></PrimaryAxis><SecondaryAxis><DefinedDirection>+X</DefinedDirection><Source>ReferenceFrame</Source><SourceDirection>+X</SourceDirection><FeatureName></FeatureName></SecondaryAxis></Value></Frame></Frames>
  Square UL : sm_lib/Body Elements/Brick Solid  BrickDimensions=square_lwh  BrickDimensionsUnits=m  ExportEntireGeometry=off  InertiaType=CalculateFromGeometry  BasedOnType=Density  Density=1000  DensityUnits=kg/m^3  Mass=1  MassUnits=kg  CenterOfMass=[0 0 0]  CenterOfMassUnits=m  MomentsOfInertia=[1 1 1]  MomentsOfInertiaUnits=kg*m^2  ProductsOfInertia=[0 0 0]  ProductsOfInertiaUnits=kg*m^2  GraphicType=FromGeometry  MarkerShape=Sphere  MarkerSize=10  GraphicVisPropType=SimpleVisualProperties  GraphicDiffuseColor=[1.0 1.0 1.0]  GraphicOpacity=1.0  GraphicSpecularColor=[0.5 0.5 0.5 1.0]  GraphicAmbientColor=[0.15 0.15 0.15 1.0]  GraphicEmissiveColor=[0.0 0.0 0.0 1.0]  GraphicShininess=75  DoExposeReferenceFrame=off  SerializedFrames=<Frames><Frame><Id>Frame1</Id><Value><Name>BL</Name><Origin><Source>GeometricFeature</Source><FeatureName>+y -z curve</FeatureName></Origin><PrimaryAxis><DefinedDirection>+Z</DefinedDirection><Source>ReferenceFrame</Source><SourceDirection>+Z</SourceDirection><FeatureName></FeatureName></PrimaryAxis><SecondaryAxis><DefinedDirection>+X</DefinedDirection><Source>ReferenceFrame</Source><SourceDirection>+X</SourceDirection><FeatureName></FeatureName></SecondaryAxis></Value></Frame><Frame><Id>Frame2</Id><Value><Name>TL</Name><Origin><Source>GeometricFeature</Source><FeatureName>+x +y +z point</FeatureName></Origin><PrimaryAxis><DefinedDirection>+Z</DefinedDirection><Source>ReferenceFrame</Source><SourceDirection>+Z</SourceDirection><FeatureName></FeatureName></PrimaryAxis><SecondaryAxis><DefinedDirection>+X</DefinedDirection><Source>ReferenceFrame</Source><SourceDirection>+X</SourceDirection><FeatureName></FeatureName></SecondaryAxis></Value></Frame><Frame><Id>Frame3</Id><Value><Name>BR</Name><Origin><Source>GeometricFeature</Source><FeatureName>-y -z curve</FeatureName></Origin><PrimaryAxis><DefinedDirection>+Z</DefinedDirection><Source>ReferenceFrame</Source><SourceDirection>+Z</SourceDirection><FeatureName></FeatureName></PrimaryAxis><SecondaryAxis><DefinedDirection>+X</DefinedDirection><Source>ReferenceFrame</Source><SourceDirection>+X</SourceDirection><FeatureName></FeatureName></SecondaryAxis></Value></Frame></Frames>
  Square UR : sm_lib/Body Elements/Brick Solid  BrickDimensions=square_lwh  BrickDimensionsUnits=m  ExportEntireGeometry=off  InertiaType=CalculateFromGeometry  BasedOnType=Density  Density=1000  DensityUnits=kg/m^3  Mass=1  MassUnits=kg  CenterOfMass=[0 0 0]  CenterOfMassUnits=m  MomentsOfInertia=[1 1 1]  MomentsOfInertiaUnits=kg*m^2  ProductsOfInertia=[0 0 0]  ProductsOfInertiaUnits=kg*m^2  GraphicType=FromGeometry  MarkerShape=Sphere  MarkerSize=10  GraphicVisPropType=SimpleVisualProperties  GraphicDiffuseColor=[0.0 0.0 0.0]  GraphicOpacity=1.0  GraphicSpecularColor=[0.5 0.5 0.5 1.0]  GraphicAmbientColor=[0.15 0.15 0.15 1.0]  GraphicEmissiveColor=[0.0 0.0 0.0 1.0]  GraphicShininess=75  DoExposeReferenceFrame=off  SerializedFrames=<Frames><Frame><Id>Frame1</Id><Value><Name>BL</Name><Origin><Source>GeometricFeature</Source><FeatureName>+y -z curve</FeatureName></Origin><PrimaryAxis><DefinedDirection>+Z</DefinedDirection><Source>ReferenceFrame</Source><SourceDirection>+Z</SourceDirection><FeatureName></FeatureName></PrimaryAxis><SecondaryAxis><DefinedDirection>+X</DefinedDirection><Source>ReferenceFrame</Source><SourceDirection>+X</SourceDirection><FeatureName></FeatureName></SecondaryAxis></Value></Frame><Frame><Id>Frame2</Id><Value><Name>TL</Name><Origin><Source>GeometricFeature</Source><FeatureName>+x +y +z point</FeatureName></Origin><PrimaryAxis><DefinedDirection>+Z</DefinedDirection><Source>ReferenceFrame</Source><SourceDirection>+Z</SourceDirection><FeatureName></FeatureName></PrimaryAxis><SecondaryAxis><DefinedDirection>+X</DefinedDirection><Source>ReferenceFrame</Source><SourceDirection>+X</SourceDirection><FeatureName></FeatureName></SecondaryAxis></Value></Frame><Frame><Id>Frame3</Id><Value><Name>BR</Name><Origin><Source>GeometricFeature</Source><FeatureName>-y -z curve</FeatureName></Origin><PrimaryAxis><DefinedDirection>+Z</DefinedDirection><Source>ReferenceFrame</Source><SourceDirection>+Z</SourceDirection><FeatureName></FeatureName></PrimaryAxis><SecondaryAxis><DefinedDirection>+X</DefinedDirection><Source>ReferenceFrame</Source><SourceDirection>+X</SourceDirection><FeatureName></FeatureName></SecondaryAxis></Value></Frame></Frames>
  BL : PMIOPort  Side=Left
  BR : PMIOPort  Port=2  Side=Right
  connections:
  Square LR/LConn1 -- Square LL/LConn2
  Square LL/LConn1 -- BL/RConn1
  Square UL/LConn1 -- Square LL/RConn1
  Square UR/LConn1 -- Square LR/RConn1
  BR/RConn1 -- Square LR/LConn2
